simulink model "Controller_testing"  (R2025b)
settings: Solver=VariableStepAuto  StartTime=0.0  StopTime=10.0  RelTol=1e-3
settings Model: Creator=Admin  LastModifiedBy=Admin

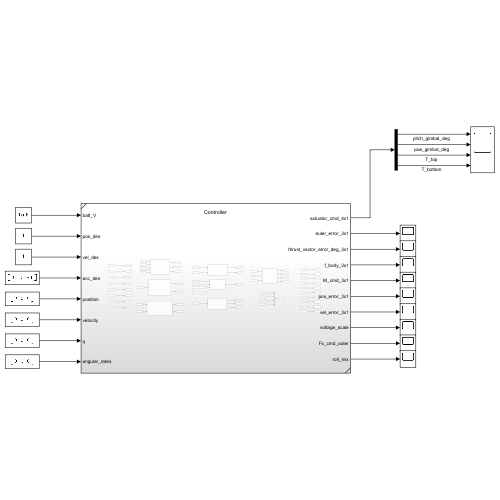
[thumbnail: Simulink's stored preview of the top-level diagram]
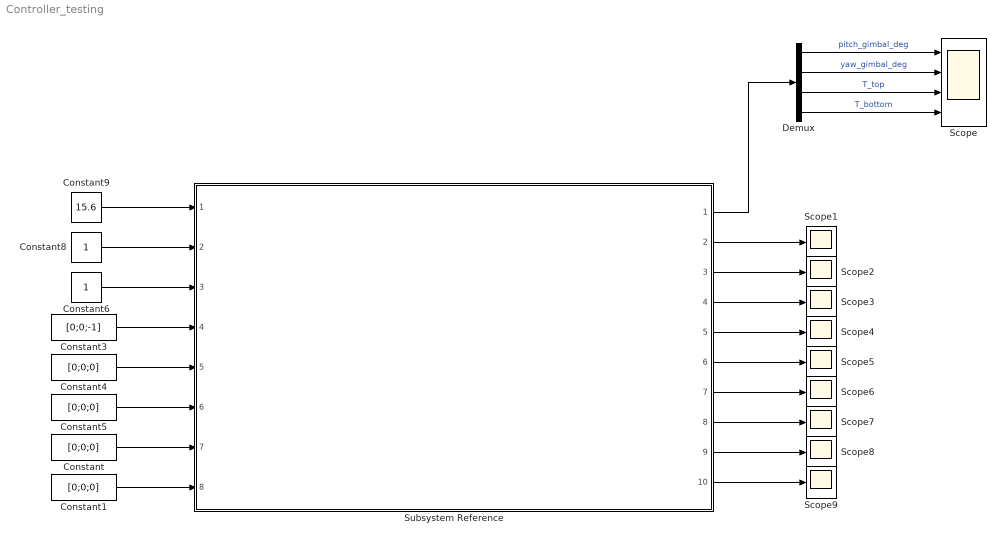
== system Controller_testing ==
  Constant{,1,4..5} (4 alike) : Constant  Value=[0;0;0]
  Constant3 : Constant  Value=[0;0;-1]
  Constant6 : Constant
  Constant8 : Constant
  Constant9 : Constant  Value=15.6
  Demux : Demux
  Scope : Scope  NumInputPorts=4
      settings: ActiveDisplayYMinimum=-150.44588186937909  ActiveDisplayYMaximum=156.28988708095949
  Scope{1..9} (9 alike) : Scope
      Scope1 settings: ActiveDisplayYMinimum=-1  ActiveDisplayYMaximum=1
      Scope2 settings: ActiveDisplayYMinimum=-1.5902773407317576E-15  ActiveDisplayYMaximum=1.4312496066585821E-14  DataLoggingVariableName=ScopeData2
      Scope3 settings: ActiveDisplayYMinimum=-1  ActiveDisplayYMaximum=1  DataLoggingVariableName=ScopeData3
      Scope4 settings: ActiveDisplayYMinimum=-1  ActiveDisplayYMaximum=1  DataLoggingVariableName=ScopeData4
      Scope5 settings: ActiveDisplayYMinimum=-1  ActiveDisplayYMaximum=1  DataLoggingVariableName=ScopeData5
      Scope6 settings: DataLoggingVariableName=ScopeData6
      Scope7 settings: DataLoggingVariableName=ScopeData7
      Scope8 settings: DataLoggingVariableName=ScopeData8
      Scope9 settings: ActiveDisplayYMinimum=-1.0032206088972568  ActiveDisplayYMaximum=26.1091757617664  DataLoggingVariableName=ScopeData9
  Subsystem Reference : Subsystem  ReferencedSubsystem=Controller
  wires:
  Subsystem Reference/2 -> Scope1/1
  Subsystem Reference/3 -> Scope2/1
  Subsystem Reference/4 -> Scope3/1
  Subsystem Reference/5 -> Scope4/1
  Subsystem Reference/6 -> Scope5/1
  Subsystem Reference/7 -> Scope6/1
  Subsystem Reference/8 -> Scope7/1
  Subsystem Reference/9 -> Scope8/1
  Subsystem Reference/10 -> Scope9/1
  Subsystem Reference/1 -> Demux/1
  Demux/2 -> Scope/2  "yaw_gimbal_deg"
  Demux/3 -> Scope/3  "T_top"
  Demux/4 -> Scope/4  "T_bottom"
  Demux/1 -> Scope/1  "pitch_gimbal_deg"
  Constant9/1 -> Subsystem Reference/1
  Constant8/1 -> Subsystem Reference/2
  Constant6/1 -> Subsystem Reference/3
  Constant3/1 -> Subsystem Reference/4
  Constant4/1 -> Subsystem Reference/5
  Constant5/1 -> Subsystem Reference/6
  Constant1/1 -> Subsystem Reference/8
  Constant/1 -> Subsystem Reference/7
